simulink model "Boost_LQR_implementation"  (R2026a)
settings: Solver=FixedStepDiscrete  StopTime=inf  FixedStep=Ts  EnableMultiTasking=on
InitFcn:
  | init_BOOT
libraries: arduinolib x2
settings Model: SILPILModeSetting=veronly  ExtModeTrigDuration=2  Creator=Usuario  LastModifiedBy=pablo_elizondo17
settings HardwareCC: ProdBitPerInt=16.0  ProdBitPerPointer=16.0  ProdBitPerSizeT=16.0  ProdBitPerPtrDiffT=16.0  ProdWordSize=8.0  ProdHWDeviceType=Atmel->AVR
settings RTWCC: SystemTargetFile=ert.tlc  HardwareBoard=Arduino Mega 2560  TLCOptions=-aInlineSetEventsForThisBaseRateFcn=TLC_FALSE -aSuppressMultiTaskScheduler=TLC_FALSE -aRateBasedStepFcn=1  Toolchain=Arduino AVR  BuildConfiguration=Faster Runs  Description=Embedded Coder
settings ERTTargetCC: ExtModeTransport=3.0  ExtModeAutomaticAllocSize=off  ExtModeStaticAllocSize=2048.0  SupportContinuousTime=on  SupportVariableSizeSignals=on

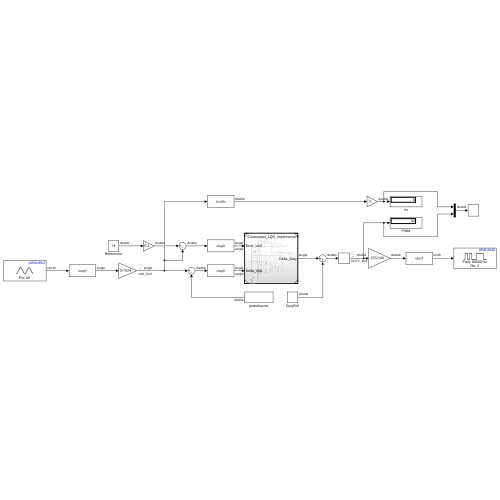
[thumbnail: Simulink's stored preview of the top-level diagram]
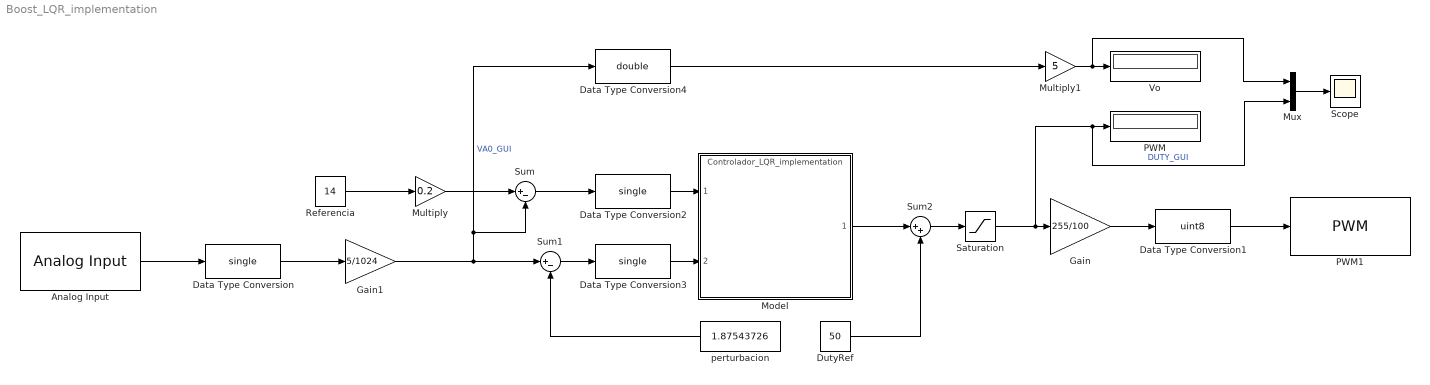
== system Boost_LQR_implementation ==
  Analog Input : arduinolib/Analog Input  pinNumber=0  ReadResultsOnly=off  ConversionTriggerSource=Software  ExternalTriggerType=uint32( 0 )  OutputDataType=uint16  EnableConversionCompleteNotify=off  EnableOuputStatus=off  SampleTime=-1  blockPlatform=arduino
      settings: LibrarySourceBlock=gizmoLibrary/Arduino Utilities/Analog Input
  Data Type Conversion : DataTypeConversion  OutDataTypeStr=single  SaturateOnIntegerOverflow=off  RndMeth=Floor
  Data Type Conversion1 : DataTypeConversion  OutDataTypeStr=uint8  SaturateOnIntegerOverflow=off  RndMeth=Floor
  Data Type Conversion2 : DataTypeConversion  OutDataTypeStr=single  SaturateOnIntegerOverflow=off  RndMeth=Floor
  Data Type Conversion3 : DataTypeConversion  OutDataTypeStr=single  SaturateOnIntegerOverflow=off  RndMeth=Floor
  Data Type Conversion4 : DataTypeConversion  OutDataTypeStr=double  SaturateOnIntegerOverflow=off  RndMeth=Floor
  DutyRef : Constant  Value=50
  Gain : Gain  Gain=255/100
  Gain1 : Gain  Gain=5/1024
  Model : ModelReference  ModelNameDialog=Controlador_LQR_implementation  SimulationMode=Normal  ModelReferenceVersion=1.3
  Multiply : Gain  Gain=0.2
  Multiply1 : Gain  Gain=5
  Mux : Mux  Inputs=2
  PWM : Display
  PWM1 : arduinolib/PWM  pinNumber=3  frequencyType=Specify  desiredFrequency=80e03  achievableFrequency=80000
      settings: LibrarySourceBlock=gizmoLibrary/Arduino Utilities/PWM
  Referencia : Constant  Value=14
  Saturation : Saturate  UpperLimit=82  LowerLimit=45
  Scope : Scope
      settings: ActiveDisplayYMinimum=10.843750000000002  ActiveDisplayYMaximum=89.90625
  Sum : Sum  Inputs=|+-
  Sum1 : Sum  Inputs=|+-
  Sum2 : Sum  Inputs=|++
  Vo : Display
  perturbacion : Constant  Value=1.87543726
  wires:
  Analog Input/1 -> Data Type Conversion/1
  Sum/1 -> Data Type Conversion2/1
  Referencia/1 -> Multiply/1
  Multiply/1 -> Sum/1
  Gain1/1 -> Data Type Conversion4/1, Sum/2, Sum1/1  "VA0_GUI"
  Sum1/1 -> Data Type Conversion3/1
  perturbacion/1 -> Sum1/2
  Saturation/1 -> Mux/2, PWM/1, Gain/1  "DUTY_GUI"
  Gain/1 -> Data Type Conversion1/1
  Data Type Conversion1/1 -> PWM1/1
  Data Type Conversion2/1 -> Model/1
  Data Type Conversion3/1 -> Model/2
  Data Type Conversion/1 -> Gain1/1
  Model/1 -> Sum2/1
  Sum2/1 -> Saturation/1
  DutyRef/1 -> Sum2/2
  Multiply1/1 -> Mux/1, Vo/1
  Mux/1 -> Scope/1
  Data Type Conversion4/1 -> Multiply1/1
